simulink model "microgrid_case5"  (R2026a)
settings: Solver=ode14x  FixedStep=50e-6
libraries: ee_lib x65, nesl_utility x33, fl_lib x29, simulink x2
(part 1 of 2)
settings Model: Creator=HAKAN SARI  LastModifiedBy=HAKAN SARI

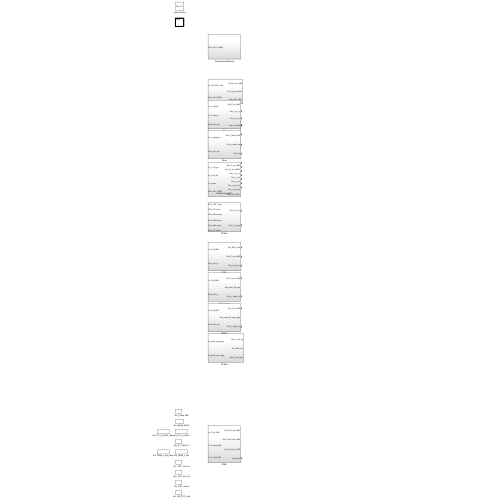
[thumbnail: Simulink's stored preview of the top-level diagram]
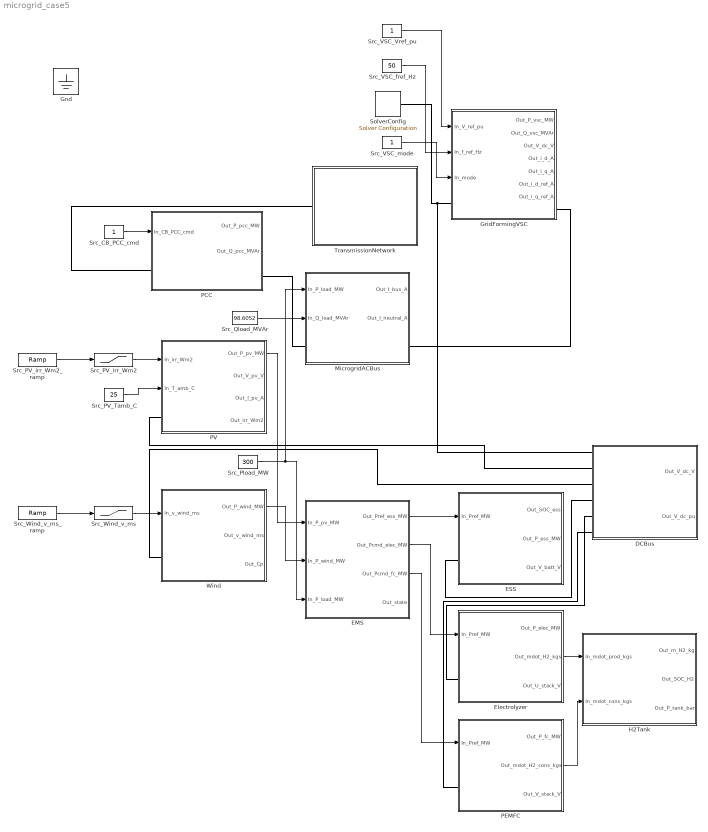
== system microgrid_case5 ==
  DCBus : Subsystem
  EMS : Subsystem
  ESS : Subsystem
  Electrolyzer : Subsystem
  Gnd : fl_lib/Electrical/Electrical Elements/Electrical Reference
  GridFormingVSC : Subsystem
  H2Tank : Subsystem
  MicrogridACBus : Subsystem
  PCC : Subsystem
  PEMFC : Subsystem
  PV : Subsystem
  SolverConfig : nesl_utility/Solver Configuration  PhysicalDomain=network_engine_domain  SubClassName=solver  LeftPortType=input  RightPortType=generic  Tones=[]  Harmonics=[]  SimulateNoise=off  Profile=off  UseLocalSampling=off  EnableSwitchedLinearOptims=on  FrequencyDomain=off  UseCCode=off  RelTol=0.001  AbsTol=0.001  MinStep=1e-09  ToWorkspace=off  RevertToSquareIcSolve=off  NumHomotopyIterations=100  PhasorMode=off  PhasorModeNumHarmonics=1  ConsistencySolver=NEWTON_XTOL_AFTER_FTOL  CanonicalOrdering=CANONICAL  OptimizeIntermediates=OPTIMIZED  IndexReductionMethod=DerivativeReplacement  DoDC=off  ResidualTolerance=1e-09  ConsistencyTolSource=GLOBAL  ConsistencyAbsTol=0.001  ConsistencyRelTol=0.001  ConsistencyTolFactor=0.001  UseLocalSolver=off  LocalSolverChoice=NE_BACKWARD_EULER_ADVANCER  ResolveIndetEquations=on  FunctionEvalNumThread=1  LocalSolverSampleTime=0.001  DoFixedCost=off  MaxNonlinIter=3  MaxModeIter=2  ComputeImpulses=off  ImpulseIterations=2  LinearAlgebra=auto  LinearAlgebraNumThread=0  EquationFormulation=NE_TIME_EF  DelaysMemoryBudget=1024  AutomaticFiltering=on  FilteringTimeConstant=0.001  PartitionStorageMethod=AS_NEEDED  PartitionMemoryBudget=1024  PartitionMethod=ROBUST  MultibodyUseLocalSolver=off  MultibodyLocalSolverChoice=ODE1  MultibodyLocalSolverSampleTime=0.001
  Src_CB_PCC_cmd : Constant
  Src_PV_Tamb_C : Constant  Value=25
  Src_PV_irr_Wm2 : Saturate  UpperLimit=800  LowerLimit=0
  Src_PV_irr_Wm2_ramp : simulink/Sources/Ramp  slope=800  start=0  InitialOutput=0
  Src_Pload_MW : Constant  Value=300
  Src_Qload_MVAr : Constant  Value=98.6052
  Src_VSC_Vref_pu : Constant
  Src_VSC_fref_Hz : Constant  Value=50
  Src_VSC_mode : Constant
  Src_Wind_v_ms : Saturate  UpperLimit=9  LowerLimit=0
  Src_Wind_v_ms_ramp : simulink/Sources/Ramp  slope=9  start=0  InitialOutput=0
  TransmissionNetwork : Subsystem
  Wind : Subsystem
  wires:
  Src_Wind_v_ms/1 -> Wind/1(In_v_wind_ms)
  Src_PV_irr_Wm2_ramp/1 -> Src_PV_irr_Wm2/1
  Src_VSC_mode/1 -> GridFormingVSC/3(In_mode)
  Src_Wind_v_ms_ramp/1 -> Src_Wind_v_ms/1
  Src_CB_PCC_cmd/1 -> PCC/1(In_CB_PCC_cmd)
  Src_PV_irr_Wm2/1 -> PV/1(In_irr_Wm2)
  Src_PV_Tamb_C/1 -> PV/2(In_T_amb_C)
  EMS/3(Out_Pcmd_fc_MW) -> PEMFC/1(In_Pref_MW)
  Src_Qload_MVAr/1 -> MicrogridACBus/2(In_Q_load_MVAr)
  PV/1(Out_P_pv_MW) -> EMS/1(In_P_pv_MW)
  Src_Pload_MW/1 -> MicrogridACBus/1(In_P_load_MW), EMS/3(In_P_load_MW)
  Wind/1(Out_P_wind_MW) -> EMS/2(In_P_wind_MW)
  Src_VSC_Vref_pu/1 -> GridFormingVSC/1(In_V_ref_pu)
  Src_VSC_fref_Hz/1 -> GridFormingVSC/2(In_f_ref_Hz)
  EMS/1(Out_Pref_ess_MW) -> ESS/1(In_Pref_MW)
  EMS/2(Out_Pcmd_elec_MW) -> Electrolyzer/1(In_Pref_MW)
  Electrolyzer/2(Out_mdot_H2_kgs) -> H2Tank/1(In_mdot_prod_kgs)
  PEMFC/2(Out_mdot_H2_cons_kgs) -> H2Tank/2(In_mdot_cons_kgs)
  connections:
  PEMFC/LConn1 -- DCBus/LConn6
  PV/LConn1 -- DCBus/LConn2
  MicrogridACBus/RConn1 -- GridFormingVSC/RConn1
  Wind/LConn1 -- DCBus/LConn3
  PCC/RConn1 -- MicrogridACBus/LConn1
  TransmissionNetwork/LConn1 -- PCC/LConn1
  SolverConfig/RConn1 -- GridFormingVSC/LConn1 -- DCBus/LConn1
  ESS/LConn1 -- DCBus/LConn4
  Electrolyzer/LConn1 -- DCBus/LConn5

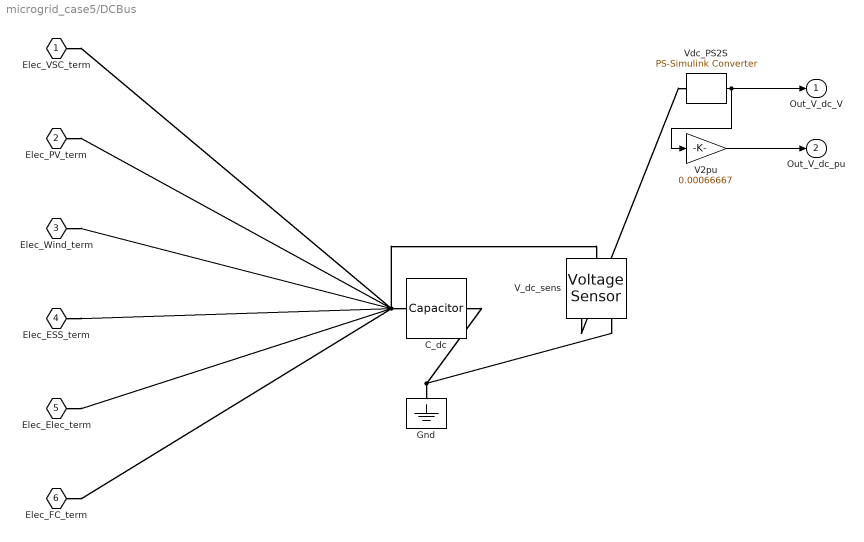
== system microgrid_case5/DCBus ==
  C_dc : ee_lib/Passive/Capacitor  cap_option=ee.enum.passive.capacitor.capOption.const  c=0.03 F  Cvec=[1e-05, 1e-06] F  Vvec=[0, 10] V  CV_table_symmetry=ee.enum.passive.capacitor.tableSymmetry.yes  f_vec=[1, 10] kHz  DFext_vec=[.8, 1.2]  enable_C_tol=ee.enum.toleranceApplication.none  averaging_period=0 s  C_tol=5  tol_distribution=ee.enum.toleranceDistribution.uniform  nSigma=4  r=0.001 Ohm  g=0 1/Ohm  enable_operating_limits=ee.enum.enable.no  operating_limit_action=ee.enum.passive.reportOpLim.warn  max_working_voltage_range=[-25, 25] V  power_rating=1 W  maxTemperature=85 degC  thermalEnable=false  thermalMass=1 J/K  i_specify=off  i_priority=None  i=0 A  i_nominal_specify=off  i_nominal_value=1  i_nominal_unit=A  v_specify=off  v_priority=None  v=0 V  v_nominal_specify=off  v_nominal_value=1  v_nominal_unit=V  vc_specify=on  vc_priority=High  vc=1500 V  vc_nominal_specify=off  vc_nominal_value=1  vc_nominal_unit=V  T_specify=off  T_priority=None  T=298.15 K  T_nominal_specify=off  T_nominal_value=1  T_nominal_unit=K
  Gnd : fl_lib/Electrical/Electrical Elements/Electrical Reference
  V2pu : Gain  Gain=0.00066667
  V_dc_sens : fl_lib/Electrical/Electrical Sensors/Voltage Sensor
  Vdc_PS2S : nesl_utility/PS-Simulink Converter  PhysicalDomain=network_engine_domain  SubClassName=ps_output  LeftPortType=input  RightPortType=output  PseudoPeriodic=off  Frequencies=[]  VectorFormat=inherit  Unit=V  AffineConversion=off
  Elec_VSC_term : PMIOPort  Side=Left
  Elec_PV_term : PMIOPort  Port=2  Side=Left
  Elec_Wind_term : PMIOPort  Port=3  Side=Left
  Elec_ESS_term : PMIOPort  Port=4  Side=Left
  Elec_Elec_term : PMIOPort  Port=5  Side=Left
  Elec_FC_term : PMIOPort  Port=6  Side=Left
  Out_V_dc_V : Outport
  Out_V_dc_pu : Outport  Port=2
  wires:
  Vdc_PS2S/1 -> Out_V_dc_V/1, V2pu/1
  V2pu/1 -> Out_V_dc_pu/1
  connections:
  Gnd/LConn1 -- C_dc/RConn1 -- V_dc_sens/RConn2
  Elec_VSC_term/RConn1 -- Elec_PV_term/RConn1 -- Elec_Wind_term/RConn1 -- Elec_ESS_term/RConn1 -- Elec_Elec_term/RConn1 -- Elec_FC_term/RConn1 -- C_dc/LConn1 -- V_dc_sens/LConn1
  V_dc_sens/RConn1 -- Vdc_PS2S/LConn1

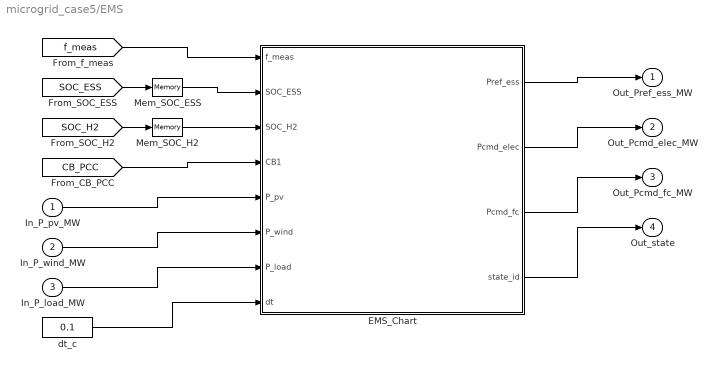
== system microgrid_case5/EMS ==
  In_P_pv_MW : Inport
  In_P_wind_MW : Inport  Port=2
  In_P_load_MW : Inport  Port=3
  EMS_Chart : Stateflow chart  TreatAsAtomicUnit=on
  Mem_SOC_ESS : Memory  InitialCondition=0.6
  Mem_SOC_H2 : Memory  InitialCondition=0.5
  dt_c : Constant  Value=0.1
  Out_Pref_ess_MW : Outport
  Out_Pcmd_elec_MW : Outport  Port=2
  Out_Pcmd_fc_MW : Outport  Port=3
  Out_state : Outport  Port=4
  wires:
  [f_meas] -> EMS_Chart/1(f_meas)
  [SOC_ESS] -> Mem_SOC_ESS/1
  Mem_SOC_ESS/1 -> EMS_Chart/2(SOC_ESS)
  [SOC_H2] -> Mem_SOC_H2/1
  Mem_SOC_H2/1 -> EMS_Chart/3(SOC_H2)
  [CB_PCC] -> EMS_Chart/4(CB1)
  In_P_pv_MW/1 -> EMS_Chart/5(P_pv)
  In_P_wind_MW/1 -> EMS_Chart/6(P_wind)
  In_P_load_MW/1 -> EMS_Chart/7(P_load)
  dt_c/1 -> EMS_Chart/8(dt)
  EMS_Chart/1(Pref_ess) -> Out_Pref_ess_MW/1
  EMS_Chart/2(Pcmd_elec) -> Out_Pcmd_elec_MW/1
  EMS_Chart/3(Pcmd_fc) -> Out_Pcmd_fc_MW/1
  EMS_Chart/4(state_id) -> Out_state/1

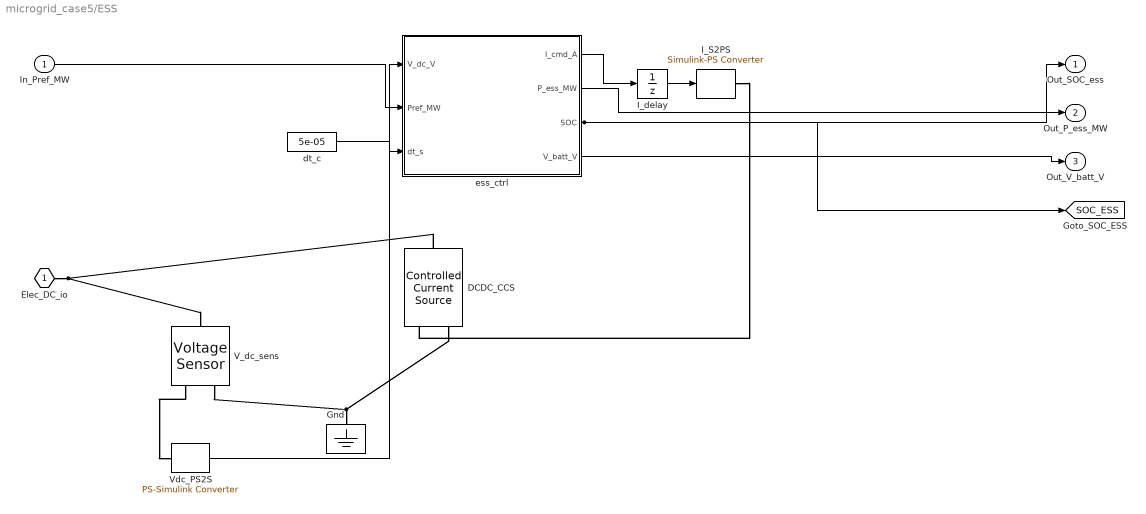
== system microgrid_case5/ESS ==
  In_Pref_MW : Inport
  DCDC_CCS : fl_lib/Electrical/Electrical Sources/Controlled Current Source
  Gnd : fl_lib/Electrical/Electrical Elements/Electrical Reference
  I_S2PS : nesl_utility/Simulink-PS Converter  PhysicalDomain=network_engine_domain  SubClassName=ps_input  LeftPortType=input  RightPortType=output  PseudoPeriodic=off  Frequencies=[]  NoiseDistribution=none  NoiseParameters=[]  Unit=A  AffineConversion=off  FilteringAndDerivatives=filter  SimscapeFilterOrder=1  InputFilterTimeConstant=1e-4  UdotUserProvided=0
  I_delay : UnitDelay  SampleTime=5e-05
  V_dc_sens : fl_lib/Electrical/Electrical Sensors/Voltage Sensor
  Vdc_PS2S : nesl_utility/PS-Simulink Converter  PhysicalDomain=network_engine_domain  SubClassName=ps_output  LeftPortType=input  RightPortType=output  PseudoPeriodic=off  Frequencies=[]  VectorFormat=inherit  Unit=V  AffineConversion=off
  dt_c : Constant  Value=5e-05
  ess_ctrl : MATLAB Function  TreatAsAtomicUnit=on
  Elec_DC_io : PMIOPort  Side=Left
  Out_SOC_ess : Outport
  Out_P_ess_MW : Outport  Port=2
  Out_V_batt_V : Outport  Port=3
  tag scope: SOC_ESS=global
  wires:
  Vdc_PS2S/1 -> ess_ctrl/1(V_dc_V)
  In_Pref_MW/1 -> ess_ctrl/2(Pref_MW)
  dt_c/1 -> ess_ctrl/3(dt_s)
  ess_ctrl/1(I_cmd_A) -> I_delay/1
  I_delay/1 -> I_S2PS/1
  ess_ctrl/2(P_ess_MW) -> Out_P_ess_MW/1
  ess_ctrl/3(SOC) -> Out_SOC_ess/1, [SOC_ESS]
  ess_ctrl/4(V_batt_V) -> Out_V_batt_V/1
  connections:
  V_dc_sens/LConn1 -- Elec_DC_io/RConn1 -- DCDC_CCS/LConn1
  Gnd/LConn1 -- V_dc_sens/RConn2 -- DCDC_CCS/RConn2
  V_dc_sens/RConn1 -- Vdc_PS2S/LConn1
  I_S2PS/RConn1 -- DCDC_CCS/RConn1

== system microgrid_case5/Electrolyzer ==
  In_Pref_MW : Inport
  EL_CCS : fl_lib/Electrical/Electrical Sources/Controlled Current Source
  Gnd : fl_lib/Electrical/Electrical Elements/Electrical Reference
  I_S2PS : nesl_utility/Simulink-PS Converter  PhysicalDomain=network_engine_domain  SubClassName=ps_input  LeftPortType=input  RightPortType=output  PseudoPeriodic=off  Frequencies=[]  NoiseDistribution=none  NoiseParameters=[]  Unit=A  AffineConversion=off  FilteringAndDerivatives=filter  SimscapeFilterOrder=1  InputFilterTimeConstant=1e-4  UdotUserProvided=0
  I_delay : UnitDelay  SampleTime=5e-05
  V_dc_sens : fl_lib/Electrical/Electrical Sensors/Voltage Sensor
  Vdc_PS2S : nesl_utility/PS-Simulink Converter  PhysicalDomain=network_engine_domain  SubClassName=ps_output  LeftPortType=input  RightPortType=output  PseudoPeriodic=off  Frequencies=[]  VectorFormat=inherit  Unit=V  AffineConversion=off
  dt_c : Constant  Value=5e-05
  el_ctrl : MATLAB Function  TreatAsAtomicUnit=on
  Elec_DC_in : PMIOPort  Side=Left
  Out_P_elec_MW : Outport
  Out_mdot_H2_kgs : Outport  Port=2
  Out_U_stack_V : Outport  Port=3
  wires:
  In_Pref_MW/1 -> el_ctrl/1(Pref_MW)
  Vdc_PS2S/1 -> el_ctrl/2(V_dc_V)
  dt_c/1 -> el_ctrl/3(dt_s)
  el_ctrl/2(P_elec_MW) -> Out_P_elec_MW/1
  el_ctrl/3(mdot_H2_kgs) -> Out_mdot_H2_kgs/1
  el_ctrl/4(U_stack_V) -> Out_U_stack_V/1
  el_ctrl/1(I_cmd_A) -> I_delay/1
  I_delay/1 -> I_S2PS/1
  connections:
  V_dc_sens/LConn1 -- Elec_DC_in/RConn1 -- EL_CCS/LConn1
  Gnd/LConn1 -- V_dc_sens/RConn2 -- EL_CCS/RConn2
  V_dc_sens/RConn1 -- Vdc_PS2S/LConn1
  I_S2PS/RConn1 -- EL_CCS/RConn1

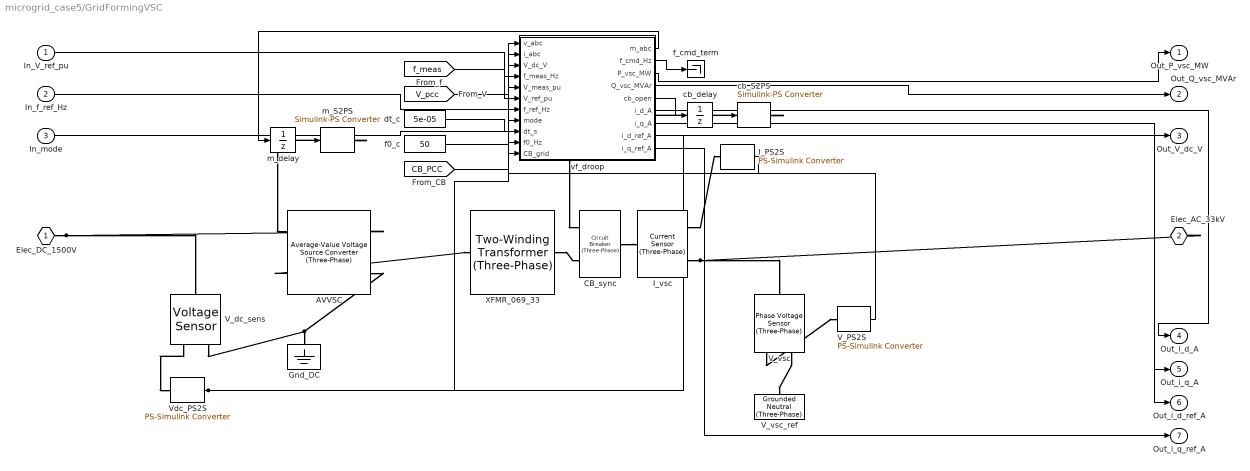
== system microgrid_case5/GridFormingVSC ==
  In_V_ref_pu : Inport
  In_f_ref_Hz : Inport  Port=2
  In_mode : Inport  Port=3
  AVVSC : ee_lib/Semiconductors & Converters/Converters/Average-Value Voltage Source Converter (Three-Phase)  port_option=ee.enum.threePhasePort.composite  enable_block_pulses_input=false  krec=0.01 Ohm  frequency_option=ee.enum.converters.frequency.variable  input_option=ee.enum.converters.inputOption.ModWave  FRated=50 Hz  losses_parameterization=ee.enum.converters.losses.fixed  Pfixed=1 W  ks=0.01  kc1=1.7 V  kc2=0.01 Ohm  Ploss_vect=[100, 800, 1870, 3250, 4900] W  Irms_vect=[10, 100, 200, 300, 400] A  Vdc_nom=1500 V  thermal_mass=30000 J/K  temperature_specify=off  temperature_priority=High  temperature=298.15 K  temperature_nominal_specify=off  temperature_nominal_value=1  temperature_nominal_unit=K
  CB_sync : ee_lib/Switches & Breakers/Circuit Breaker (Three-Phase)  port_option=ee.enum.threePhasePort.composite  control_port_option=ee.enum.controlport.ps  R_closed=1e-3 Ohm  G_open=1e-6 1/Ohm  threshold=0.5 V  breaker_behavior=ee.enum.switches.breakerBehavior.zeroCrossingEnable  i_th=1e-8 A
  Gnd_DC : fl_lib/Electrical/Electrical Elements/Electrical Reference
  I_PS2S : nesl_utility/PS-Simulink Converter  PhysicalDomain=network_engine_domain  SubClassName=ps_output  LeftPortType=input  RightPortType=output  PseudoPeriodic=off  Frequencies=[]  VectorFormat=inherit  Unit=inherit  AffineConversion=off
  I_vsc : ee_lib/Sensors & Transducers/Current Sensor (Three-Phase)  port_option=ee.enum.threePhasePort.composite
  V_PS2S : nesl_utility/PS-Simulink Converter  PhysicalDomain=network_engine_domain  SubClassName=ps_output  LeftPortType=input  RightPortType=output  PseudoPeriodic=off  Frequencies=[]  VectorFormat=inherit  Unit=inherit  AffineConversion=off
  V_dc_sens : fl_lib/Electrical/Electrical Sensors/Voltage Sensor
  V_vsc : ee_lib/Sensors & Transducers/Phase Voltage Sensor (Three-Phase)  port_option=ee.enum.threePhasePort.composite
  V_vsc_ref : ee_lib/Connectors & References/Grounded Neutral (Three-Phase)  port_option=ee.enum.threePhasePort.composite
  Vdc_PS2S : nesl_utility/PS-Simulink Converter  PhysicalDomain=network_engine_domain  SubClassName=ps_output  LeftPortType=input  RightPortType=output  PseudoPeriodic=off  Frequencies=[]  VectorFormat=inherit  Unit=V  AffineConversion=off
  XFMR_069_33 : ee_lib/Passive/Transformers/Two-Winding Transformer (Three-Phase)  SRated=350000000 A*V  FRated=50 Hz  Winding1Connection=ee.enum.windingconnection.Yg  VRated1=690 V  Winding2Connection=ee.enum.windingconnection.delta11  VRated2=33000 V  CoreType=ee.enum.coretype.threelimb  pu_Rw1=0.002  pu_Rw2=0.002  leakage_reactance_option=ee.enum.transformer_leakage.include  pu_Xl1=0.05  pu_Xl2=0.05  magnetizing_resistance_option=ee.enum.transformer_magnetizingResistance.exclude  pu_Rm=500  magnetizing_reactance_option=ee.enum.transformer_magnetizingReactance.exclude  saturation_option=ee.enum.transformer_saturation.exclude  pu_Xm=500  current_data=[0, .002, 1, 2]  magnetic_flux_data=[0, 1.2, 1.5, 1.51]  pu_X0=0.5  i1_specify=off  i1_priority=None  i1=[0, 0, 0] A  i1_nominal_specify=off  i1_nominal_value=1  i1_nominal_unit=A  i2_specify=off  i2_priority=None  i2=[0, 0, 0] A  i2_nominal_specify=off  i2_nominal_value=1  i2_nominal_unit=A  phi_specify=off  phi_priority=None  phi=[0, 0, 0]  phi_nominal_specify=off  phi_nominal_value=1  phi_nominal_unit=1
  cb_S2PS : nesl_utility/Simulink-PS Converter  PhysicalDomain=network_engine_domain  SubClassName=ps_input  LeftPortType=input  RightPortType=output  PseudoPeriodic=off  Frequencies=[]  NoiseDistribution=none  NoiseParameters=[]  Unit=1  AffineConversion=off  FilteringAndDerivatives=provide  SimscapeFilterOrder=1  InputFilterTimeConstant=0.001  UdotUserProvided=0
  cb_delay : UnitDelay  InitialCondition=1  SampleTime=5e-05
  dt_c : Constant  Value=5e-05
  f0_c : Constant  Value=50
  f_cmd_term : Terminator
  m_S2PS : nesl_utility/Simulink-PS Converter  PhysicalDomain=network_engine_domain  SubClassName=ps_input  LeftPortType=input  RightPortType=output  PseudoPeriodic=off  Frequencies=[]  NoiseDistribution=none  NoiseParameters=[]  Unit=1  AffineConversion=off  FilteringAndDerivatives=filter  SimscapeFilterOrder=1  InputFilterTimeConstant=1e-4  UdotUserProvided=0
  m_delay : UnitDelay  SampleTime=5e-05
  vf_droop : MATLAB Function  TreatAsAtomicUnit=on
  Elec_DC_1500V : PMIOPort  Side=Left
  Elec_AC_33kV : PMIOPort  Port=2  Side=Right
  Out_P_vsc_MW : Outport
  Out_Q_vsc_MVAr : Outport  Port=2
  Out_V_dc_V : Outport  Port=3
  Out_i_d_A : Outport  Port=4
  Out_i_q_A : Outport  Port=5
  Out_i_d_ref_A : Outport  Port=6
  Out_i_q_ref_A : Outport  Port=7
  wires:
  Vdc_PS2S/1 -> Out_V_dc_V/1, vf_droop/3(V_dc_V)
  V_PS2S/1 -> vf_droop/1(v_abc)
  I_PS2S/1 -> vf_droop/2(i_abc)
  [f_meas] -> vf_droop/4(f_meas_Hz)
  [V_pcc] -> vf_droop/5(V_meas_pu)
  In_V_ref_pu/1 -> vf_droop/6(V_ref_pu)
  In_f_ref_Hz/1 -> vf_droop/7(f_ref_Hz)
  In_mode/1 -> vf_droop/8(mode)
  dt_c/1 -> vf_droop/9(dt_s)
  f0_c/1 -> vf_droop/10(f0_Hz)
  [CB_PCC] -> vf_droop/11(CB_grid)
  vf_droop/1(m_abc) -> m_delay/1
  m_delay/1 -> m_S2PS/1
  vf_droop/2(f_cmd_Hz) -> f_cmd_term/1
  vf_droop/3(P_vsc_MW) -> Out_P_vsc_MW/1
  vf_droop/4(Q_vsc_MVAr) -> Out_Q_vsc_MVAr/1
  vf_droop/6(i_d_A) -> Out_i_d_A/1
  vf_droop/7(i_q_A) -> Out_i_q_A/1
  vf_droop/8(i_d_ref_A) -> Out_i_d_ref_A/1
  vf_droop/9(i_q_ref_A) -> Out_i_q_ref_A/1
  vf_droop/5(cb_open) -> cb_delay/1
  cb_delay/1 -> cb_S2PS/1
  connections:
  AVVSC/RConn1 -- Elec_DC_1500V/RConn1 -- V_dc_sens/LConn1
  Gnd_DC/LConn1 -- AVVSC/RConn2 -- V_dc_sens/RConn2
  V_dc_sens/RConn1 -- Vdc_PS2S/LConn1
  AVVSC/LConn2 -- XFMR_069_33/LConn1
  XFMR_069_33/RConn1 -- CB_sync/LConn2
  CB_sync/RConn1 -- I_vsc/LConn1
  Elec_AC_33kV/RConn1 -- I_vsc/RConn2 -- V_vsc/LConn1
  V_vsc/RConn2 -- V_vsc_ref/LConn1
  I_vsc/RConn1 -- I_PS2S/LConn1
  V_vsc/RConn1 -- V_PS2S/LConn1
  m_S2PS/RConn1 -- AVVSC/LConn1
  cb_S2PS/RConn1 -- CB_sync/LConn1

== system microgrid_case5/H2Tank ==
  In_mdot_prod_kgs : Inport
  In_mdot_cons_kgs : Inport  Port=2
  dt_c : Constant  Value=5e-05
  tank_dynamics : MATLAB Function  TreatAsAtomicUnit=on
  Out_m_H2_kg : Outport
  Out_SOC_H2 : Outport  Port=2
  Out_P_tank_bar : Outport  Port=3
  tag scope: SOC_H2=global
  wires:
  In_mdot_prod_kgs/1 -> tank_dynamics/1(mdot_prod_kgs)
  In_mdot_cons_kgs/1 -> tank_dynamics/2(mdot_cons_kgs)
  dt_c/1 -> tank_dynamics/3(dt_s)
  tank_dynamics/1(m_H2_kg) -> Out_m_H2_kg/1
  tank_dynamics/2(SOC_H2) -> Out_SOC_H2/1, [SOC_H2]
  tank_dynamics/3(P_tank_bar) -> Out_P_tank_bar/1

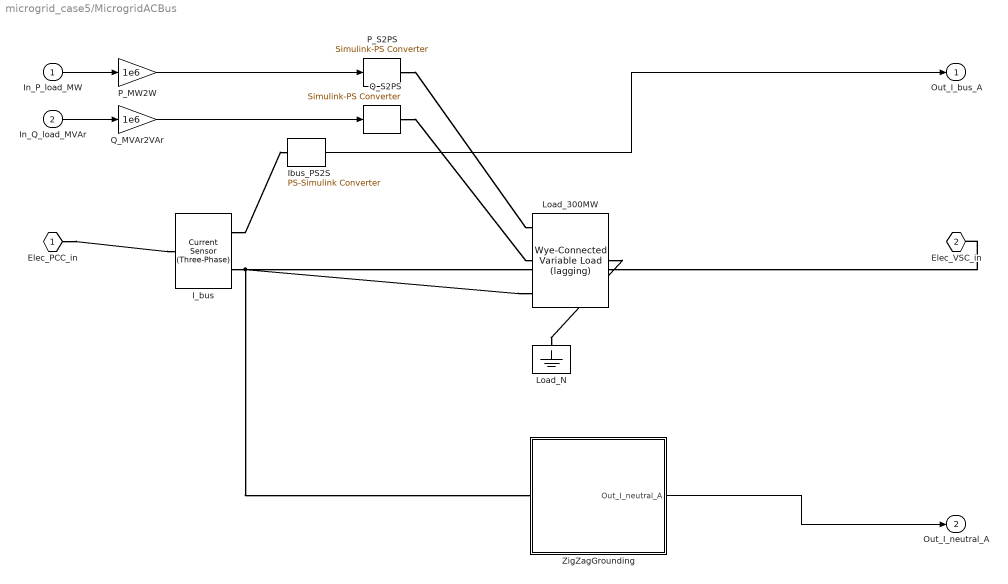
== system microgrid_case5/MicrogridACBus ==
  In_P_load_MW : Inport
  In_Q_load_MVAr : Inport  Port=2
  I_bus : ee_lib/Sensors & Transducers/Current Sensor (Three-Phase)  port_option=ee.enum.threePhasePort.composite
  Ibus_PS2S : nesl_utility/PS-Simulink Converter  PhysicalDomain=network_engine_domain  SubClassName=ps_output  LeftPortType=input  RightPortType=output  PseudoPeriodic=off  Frequencies=[]  VectorFormat=inherit  Unit=inherit  AffineConversion=off
  Load_300MW : ee_lib/Passive/RLC Assemblies/Wye-Connected Variable Load (lagging)  port_option=ee.enum.threePhasePort.composite  VRated=33000 V  FRated=50 Hz  Pmin=1e3 W  Qmin=1e3 A*V  G_parasitic=1e-6 1/Ohm  I_specify=off  I_priority=None  I=[0, 0, 0] A  I_nominal_specify=off  I_nominal_value=1  I_nominal_unit=A  Phi_specify=off  Phi_priority=None  Phi=[0, 0, 0] Wb  Phi_nominal_specify=off  Phi_nominal_value=1  Phi_nominal_unit=Wb
  Load_N : fl_lib/Electrical/Electrical Elements/Electrical Reference
  P_MW2W : Gain  Gain=1e6
  P_S2PS : nesl_utility/Simulink-PS Converter  PhysicalDomain=network_engine_domain  SubClassName=ps_input  LeftPortType=input  RightPortType=output  PseudoPeriodic=off  Frequencies=[]  NoiseDistribution=none  NoiseParameters=[]  Unit=W  AffineConversion=off  FilteringAndDerivatives=provide  SimscapeFilterOrder=1  InputFilterTimeConstant=0.001  UdotUserProvided=0
  Q_MVAr2VAr : Gain  Gain=1e6
  Q_S2PS : nesl_utility/Simulink-PS Converter  PhysicalDomain=network_engine_domain  SubClassName=ps_input  LeftPortType=input  RightPortType=output  PseudoPeriodic=off  Frequencies=[]  NoiseDistribution=none  NoiseParameters=[]  Unit=V*A  AffineConversion=off  FilteringAndDerivatives=provide  SimscapeFilterOrder=1  InputFilterTimeConstant=0.001  UdotUserProvided=0
  ZigZagGrounding : Subsystem
  Elec_PCC_in : PMIOPort  Side=Left
  Elec_VSC_in : PMIOPort  Port=2  Side=Right
  Out_I_bus_A : Outport
  Out_I_neutral_A : Outport  Port=2
  wires:
  Ibus_PS2S/1 -> Out_I_bus_A/1
  In_P_load_MW/1 -> P_MW2W/1
  P_MW2W/1 -> P_S2PS/1
  In_Q_load_MVAr/1 -> Q_MVAr2VAr/1
  Q_MVAr2VAr/1 -> Q_S2PS/1
  ZigZagGrounding/1(Out_I_neutral_A) -> Out_I_neutral_A/1
  connections:
  Elec_PCC_in/RConn1 -- I_bus/LConn1
  I_bus/RConn1 -- Ibus_PS2S/LConn1
  Load_300MW/LConn3 -- I_bus/RConn2 -- Elec_VSC_in/RConn1 -- ZigZagGrounding/LConn1
  Load_300MW/RConn1 -- Load_N/LConn1
  P_S2PS/RConn1 -- Load_300MW/LConn1
  Q_S2PS/RConn1 -- Load_300MW/LConn2

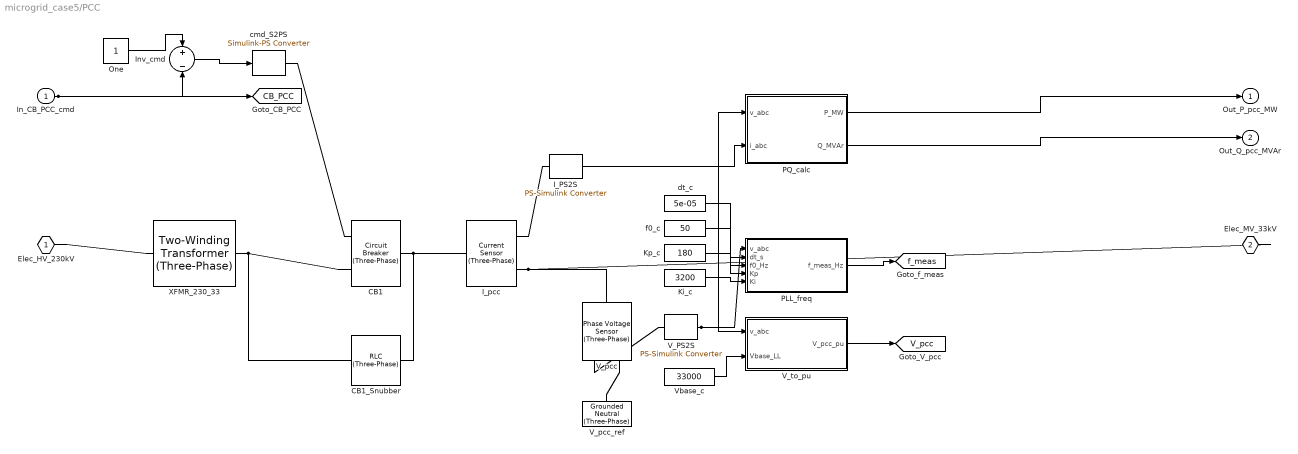
== system microgrid_case5/PCC ==
  In_CB_PCC_cmd : Inport
  CB1 : ee_lib/Switches & Breakers/Circuit Breaker (Three-Phase)  port_option=ee.enum.threePhasePort.composite  control_port_option=ee.enum.controlport.ps  R_closed=1e-3 Ohm  G_open=1e-6 1/Ohm  threshold=0.5 V  breaker_behavior=ee.enum.switches.breakerBehavior.zeroCrossingEnable  i_th=1e-8 A
  CB1_Snubber : ee_lib/Passive/RLC Assemblies/RLC (Three-Phase)  port_option=ee.enum.threePhasePort.composite  component_structure=ee.enum.rlc.structure.SeriesRC  R=200 Ohm  L=1e-3 H  C=1e-06 F  R_parasitic=0 Ohm  G_parasitic=0 1/Ohm  IL_specify=off  IL_priority=High  IL=[0, 0, 0] A  IL_nominal_specify=off  IL_nominal_value=1  IL_nominal_unit=A  VC_specify=off  VC_priority=High  VC=[0, 0, 0] V  VC_nominal_specify=off  VC_nominal_value=1  VC_nominal_unit=V
  I_PS2S : nesl_utility/PS-Simulink Converter  PhysicalDomain=network_engine_domain  SubClassName=ps_output  LeftPortType=input  RightPortType=output  PseudoPeriodic=off  Frequencies=[]  VectorFormat=inherit  Unit=inherit  AffineConversion=off
  I_pcc : ee_lib/Sensors & Transducers/Current Sensor (Three-Phase)  port_option=ee.enum.threePhasePort.composite
  Inv_cmd : Sum  Inputs=+-
  Ki_c : Constant  Value=3200
  Kp_c : Constant  Value=180
  One : Constant
  PLL_freq : MATLAB Function  TreatAsAtomicUnit=on
  PQ_calc : MATLAB Function  TreatAsAtomicUnit=on
  V_PS2S : nesl_utility/PS-Simulink Converter  PhysicalDomain=network_engine_domain  SubClassName=ps_output  LeftPortType=input  RightPortType=output  PseudoPeriodic=off  Frequencies=[]  VectorFormat=inherit  Unit=inherit  AffineConversion=off
  V_pcc : ee_lib/Sensors & Transducers/Phase Voltage Sensor (Three-Phase)  port_option=ee.enum.threePhasePort.composite
  V_pcc_ref : ee_lib/Connectors & References/Grounded Neutral (Three-Phase)  port_option=ee.enum.threePhasePort.composite
  V_to_pu : MATLAB Function  TreatAsAtomicUnit=on
  Vbase_c : Constant  Value=33000
  XFMR_230_33 : ee_lib/Passive/Transformers/Two-Winding Transformer (Three-Phase)  SRated=300000000 A*V  FRated=50 Hz  Winding1Connection=ee.enum.windingconnection.delta11  VRated1=230000 V  Winding2Connection=ee.enum.windingconnection.Yg  VRated2=33000 V  CoreType=ee.enum.coretype.threelimb  pu_Rw1=0.002  pu_Rw2=0.002  leakage_reactance_option=ee.enum.transformer_leakage.include  pu_Xl1=0.05  pu_Xl2=0.05  magnetizing_resistance_option=ee.enum.transformer_magnetizingResistance.exclude  pu_Rm=500  magnetizing_reactance_option=ee.enum.transformer_magnetizingReactance.exclude  saturation_option=ee.enum.transformer_saturation.exclude  pu_Xm=500  current_data=[0, .002, 1, 2]  magnetic_flux_data=[0, 1.2, 1.5, 1.51]  pu_X0=0.5  i1_specify=off  i1_priority=None  i1=[0, 0, 0] A  i1_nominal_specify=off  i1_nominal_value=1  i1_nominal_unit=A  i2_specify=off  i2_priority=None  i2=[0, 0, 0] A  i2_nominal_specify=off  i2_nominal_value=1  i2_nominal_unit=A  phi_specify=off  phi_priority=None  phi=[0, 0, 0]  phi_nominal_specify=off  phi_nominal_value=1  phi_nominal_unit=1
  cmd_S2PS : nesl_utility/Simulink-PS Converter  PhysicalDomain=network_engine_domain  SubClassName=ps_input  LeftPortType=input  RightPortType=output  PseudoPeriodic=off  Frequencies=[]  NoiseDistribution=none  NoiseParameters=[]  Unit=1  AffineConversion=off  FilteringAndDerivatives=filter  SimscapeFilterOrder=1  InputFilterTimeConstant=1e-4  UdotUserProvided=0
  dt_c : Constant  Value=5e-05
  f0_c : Constant  Value=50
  Elec_HV_230kV : PMIOPort  Side=Left
  Elec_MV_33kV : PMIOPort  Port=2  Side=Right
  Out_P_pcc_MW : Outport
  Out_Q_pcc_MVAr : Outport  Port=2
  tag scope: CB_PCC=global, V_pcc=global, f_meas=global
  wires:
  One/1 -> Inv_cmd/1
  In_CB_PCC_cmd/1 -> Inv_cmd/2, [CB_PCC]
  Inv_cmd/1 -> cmd_S2PS/1
  V_PS2S/1 -> PLL_freq/1(v_abc), V_to_pu/1(v_abc), PQ_calc/1(v_abc)
  dt_c/1 -> PLL_freq/2(dt_s)
  f0_c/1 -> PLL_freq/3(f0_Hz)
  Kp_c/1 -> PLL_freq/4(Kp)
  Ki_c/1 -> PLL_freq/5(Ki)
  PLL_freq/1(f_meas_Hz) -> [f_meas]
  Vbase_c/1 -> V_to_pu/2(Vbase_LL)
  V_to_pu/1(V_pcc_pu) -> [V_pcc]
  I_PS2S/1 -> PQ_calc/2(i_abc)
  PQ_calc/1(P_MW) -> Out_P_pcc_MW/1
  PQ_calc/2(Q_MVAr) -> Out_Q_pcc_MVAr/1
  connections:
  Elec_HV_230kV/RConn1 -- XFMR_230_33/LConn1
  CB1/LConn2 -- XFMR_230_33/RConn1 -- CB1_Snubber/LConn1
  cmd_S2PS/RConn1 -- CB1/LConn1
  CB1_Snubber/RConn1 -- CB1/RConn1 -- I_pcc/LConn1
  Elec_MV_33kV/RConn1 -- I_pcc/RConn2 -- V_pcc/LConn1
  V_pcc/RConn2 -- V_pcc_ref/LConn1
  I_pcc/RConn1 -- I_PS2S/LConn1
  V_pcc/RConn1 -- V_PS2S/LConn1

== system microgrid_case5/PEMFC ==
  In_Pref_MW : Inport
  FC_CCS : fl_lib/Electrical/Electrical Sources/Controlled Current Source
  Gnd : fl_lib/Electrical/Electrical Elements/Electrical Reference
  I_S2PS : nesl_utility/Simulink-PS Converter  PhysicalDomain=network_engine_domain  SubClassName=ps_input  LeftPortType=input  RightPortType=output  PseudoPeriodic=off  Frequencies=[]  NoiseDistribution=none  NoiseParameters=[]  Unit=A  AffineConversion=off  FilteringAndDerivatives=filter  SimscapeFilterOrder=1  InputFilterTimeConstant=1e-4  UdotUserProvided=0
  I_delay : UnitDelay  SampleTime=5e-05
  V_dc_sens : fl_lib/Electrical/Electrical Sensors/Voltage Sensor
  Vdc_PS2S : nesl_utility/PS-Simulink Converter  PhysicalDomain=network_engine_domain  SubClassName=ps_output  LeftPortType=input  RightPortType=output  PseudoPeriodic=off  Frequencies=[]  VectorFormat=inherit  Unit=V  AffineConversion=off
  dt_c : Constant  Value=5e-05
  fc_ctrl : MATLAB Function  TreatAsAtomicUnit=on
  Elec_DC_out : PMIOPort  Side=Left
  Out_P_fc_MW : Outport
  Out_mdot_H2_cons_kgs : Outport  Port=2
  Out_V_stack_V : Outport  Port=3
  wires:
  In_Pref_MW/1 -> fc_ctrl/1(Pref_MW)
  Vdc_PS2S/1 -> fc_ctrl/2(V_dc_V)
  dt_c/1 -> fc_ctrl/3(dt_s)
  fc_ctrl/2(P_fc_MW) -> Out_P_fc_MW/1
  fc_ctrl/3(mdot_cons_kgs) -> Out_mdot_H2_cons_kgs/1
  fc_ctrl/4(V_stack_V) -> Out_V_stack_V/1
  fc_ctrl/1(I_cmd_A) -> I_delay/1
  I_delay/1 -> I_S2PS/1
  connections:
  V_dc_sens/LConn1 -- Elec_DC_out/RConn1 -- FC_CCS/LConn1
  Gnd/LConn1 -- V_dc_sens/RConn2 -- FC_CCS/RConn2
  V_dc_sens/RConn1 -- Vdc_PS2S/LConn1
  I_S2PS/RConn1 -- FC_CCS/RConn1

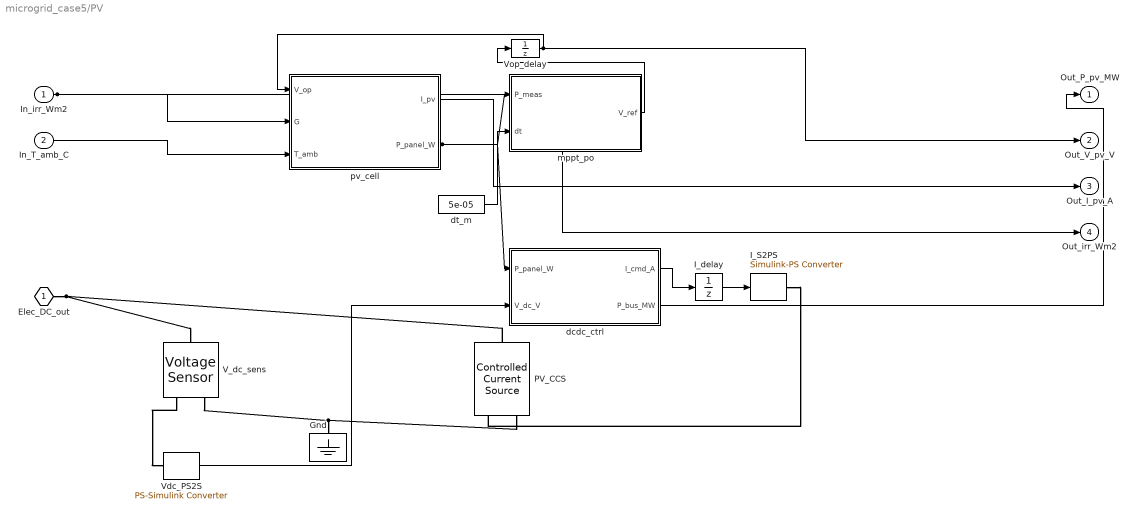
== system microgrid_case5/PV ==
  In_irr_Wm2 : Inport
  In_T_amb_C : Inport  Port=2
  Gnd : fl_lib/Electrical/Electrical Elements/Electrical Reference
  I_S2PS : nesl_utility/Simulink-PS Converter  PhysicalDomain=network_engine_domain  SubClassName=ps_input  LeftPortType=input  RightPortType=output  PseudoPeriodic=off  Frequencies=[]  NoiseDistribution=none  NoiseParameters=[]  Unit=A  AffineConversion=off  FilteringAndDerivatives=filter  SimscapeFilterOrder=1  InputFilterTimeConstant=1e-4  UdotUserProvided=0
  I_delay : UnitDelay  SampleTime=5e-05
  PV_CCS : fl_lib/Electrical/Electrical Sources/Controlled Current Source
  V_dc_sens : fl_lib/Electrical/Electrical Sensors/Voltage Sensor
  Vdc_PS2S : nesl_utility/PS-Simulink Converter  PhysicalDomain=network_engine_domain  SubClassName=ps_output  LeftPortType=input  RightPortType=output  PseudoPeriodic=off  Frequencies=[]  VectorFormat=inherit  Unit=V  AffineConversion=off
  Vop_delay : UnitDelay  InitialCondition=702  SampleTime=5e-05
  dcdc_ctrl : MATLAB Function  TreatAsAtomicUnit=on
  dt_m : Constant  Value=5e-05
  mppt_po : MATLAB Function  TreatAsAtomicUnit=on
  pv_cell : MATLAB Function  TreatAsAtomicUnit=on
  Elec_DC_out : PMIOPort  Side=Left
  Out_P_pv_MW : Outport
  Out_V_pv_V : Outport  Port=2
  Out_I_pv_A : Outport  Port=3
  Out_irr_Wm2 : Outport  Port=4
  wires:
  In_irr_Wm2/1 -> Out_irr_Wm2/1, pv_cell/2(G)
  In_T_amb_C/1 -> pv_cell/3(T_amb)
  pv_cell/2(P_panel_W) -> mppt_po/1(P_meas), dcdc_ctrl/1(P_panel_W)
  dt_m/1 -> mppt_po/2(dt)
  mppt_po/1(V_ref) -> Vop_delay/1
  Vop_delay/1 -> pv_cell/1(V_op), Out_V_pv_V/1
  pv_cell/1(I_pv) -> Out_I_pv_A/1
  Vdc_PS2S/1 -> dcdc_ctrl/2(V_dc_V)
  dcdc_ctrl/2(P_bus_MW) -> Out_P_pv_MW/1
  dcdc_ctrl/1(I_cmd_A) -> I_delay/1
  I_delay/1 -> I_S2PS/1
  connections:
  V_dc_sens/LConn1 -- Elec_DC_out/RConn1 -- PV_CCS/LConn1
  Gnd/LConn1 -- V_dc_sens/RConn2 -- PV_CCS/RConn2
  V_dc_sens/RConn1 -- Vdc_PS2S/LConn1
  I_S2PS/RConn1 -- PV_CCS/RConn1

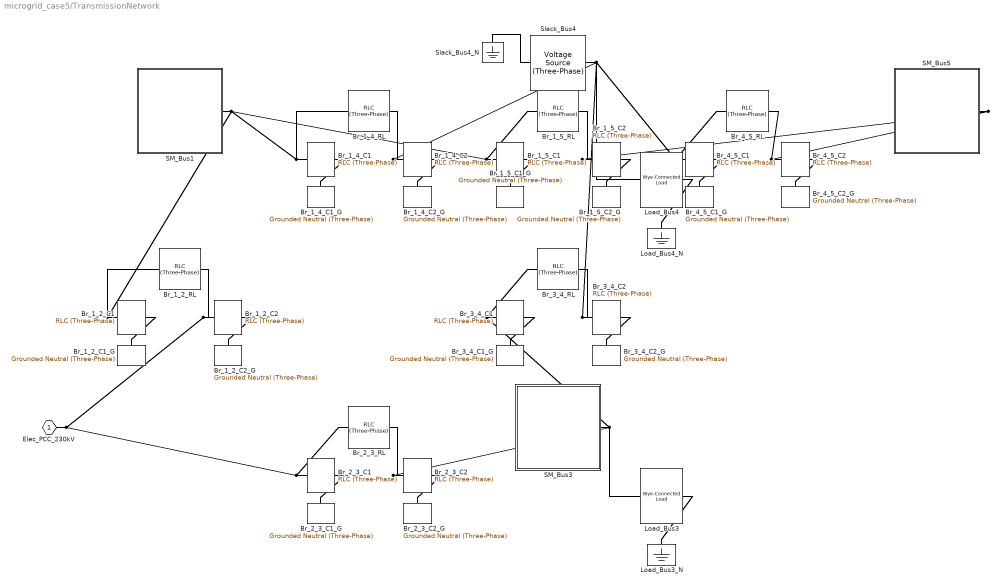
== system microgrid_case5/TransmissionNetwork ==
  Br_1_2_C1 : ee_lib/Passive/RLC Assemblies/RLC (Three-Phase)  port_option=ee.enum.threePhasePort.composite  component_structure=ee.enum.rlc.structure.C  R=1 Ohm  L=1e-3 H  C=2.1421e-08 F  R_parasitic=1 Ohm  G_parasitic=0 1/Ohm  IL_specify=off  IL_priority=High  IL=[0, 0, 0] A  IL_nominal_specify=off  IL_nominal_value=1  IL_nominal_unit=A  VC_specify=off  VC_priority=High  VC=[0, 0, 0] V  VC_nominal_specify=off  VC_nominal_value=1  VC_nominal_unit=V
  Br_1_2_C1_G : ee_lib/Connectors & References/Grounded Neutral (Three-Phase)  port_option=ee.enum.threePhasePort.composite
  Br_1_2_C2 : ee_lib/Passive/RLC Assemblies/RLC (Three-Phase)  port_option=ee.enum.threePhasePort.composite  component_structure=ee.enum.rlc.structure.C  R=1 Ohm  L=1e-3 H  C=2.1421e-08 F  R_parasitic=1 Ohm  G_parasitic=0 1/Ohm  IL_specify=off  IL_priority=High  IL=[0, 0, 0] A  IL_nominal_specify=off  IL_nominal_value=1  IL_nominal_unit=A  VC_specify=off  VC_priority=High  VC=[0, 0, 0] V  VC_nominal_specify=off  VC_nominal_value=1  VC_nominal_unit=V
  Br_1_2_C2_G : ee_lib/Connectors & References/Grounded Neutral (Three-Phase)  port_option=ee.enum.threePhasePort.composite
  Br_1_2_RL : ee_lib/Passive/RLC Assemblies/RLC (Three-Phase)  port_option=ee.enum.threePhasePort.composite  component_structure=ee.enum.rlc.structure.SeriesRL  R=1.4865 Ohm  L=0.047316 H  C=1e-6 F  R_parasitic=0 Ohm  G_parasitic=0 1/Ohm  IL_specify=off  IL_priority=High  IL=[0, 0, 0] A  IL_nominal_specify=off  IL_nominal_value=1  IL_nominal_unit=A  VC_specify=off  VC_priority=High  VC=[0, 0, 0] V  VC_nominal_specify=off  VC_nominal_value=1  VC_nominal_unit=V
  Br_1_4_C1 : ee_lib/Passive/RLC Assemblies/RLC (Three-Phase)  port_option=ee.enum.threePhasePort.composite  component_structure=ee.enum.rlc.structure.C  R=1 Ohm  L=1e-3 H  C=1.9797e-08 F  R_parasitic=1 Ohm  G_parasitic=0 1/Ohm  IL_specify=off  IL_priority=High  IL=[0, 0, 0] A  IL_nominal_specify=off  IL_nominal_value=1  IL_nominal_unit=A  VC_specify=off  VC_priority=High  VC=[0, 0, 0] V  VC_nominal_specify=off  VC_nominal_value=1  VC_nominal_unit=V
  Br_1_4_C1_G : ee_lib/Connectors & References/Grounded Neutral (Three-Phase)  port_option=ee.enum.threePhasePort.composite
  Br_1_4_C2 : ee_lib/Passive/RLC Assemblies/RLC (Three-Phase)  port_option=ee.enum.threePhasePort.composite  component_structure=ee.enum.rlc.structure.C  R=1 Ohm  L=1e-3 H  C=1.9797e-08 F  R_parasitic=1 Ohm  G_parasitic=0 1/Ohm  IL_specify=off  IL_priority=High  IL=[0, 0, 0] A  IL_nominal_specify=off  IL_nominal_value=1  IL_nominal_unit=A  VC_specify=off  VC_priority=High  VC=[0, 0, 0] V  VC_nominal_specify=off  VC_nominal_value=1  VC_nominal_unit=V
  Br_1_4_C2_G : ee_lib/Connectors & References/Grounded Neutral (Three-Phase)  port_option=ee.enum.threePhasePort.composite
  Br_1_4_RL : ee_lib/Passive/RLC Assemblies/RLC (Three-Phase)  port_option=ee.enum.threePhasePort.composite  component_structure=ee.enum.rlc.structure.SeriesRL  R=1.6082 Ohm  L=0.051189 H  C=1e-6 F  R_parasitic=0 Ohm  G_parasitic=0 1/Ohm  IL_specify=off  IL_priority=High  IL=[0, 0, 0] A  IL_nominal_specify=off  IL_nominal_value=1  IL_nominal_unit=A  VC_specify=off  VC_priority=High  VC=[0, 0, 0] V  VC_nominal_specify=off  VC_nominal_value=1  VC_nominal_unit=V
  Br_1_5_C1 : ee_lib/Passive/RLC Assemblies/RLC (Three-Phase)  port_option=ee.enum.threePhasePort.composite  component_structure=ee.enum.rlc.structure.C  R=1 Ohm  L=1e-3 H  C=9.4049e-08 F  R_parasitic=1 Ohm  G_parasitic=0 1/Ohm  IL_specify=off  IL_priority=High  IL=[0, 0, 0] A  IL_nominal_specify=off  IL_nominal_value=1  IL_nominal_unit=A  VC_specify=off  VC_priority=High  VC=[0, 0, 0] V  VC_nominal_specify=off  VC_nominal_value=1  VC_nominal_unit=V
  Br_1_5_C1_G : ee_lib/Connectors & References/Grounded Neutral (Three-Phase)  port_option=ee.enum.threePhasePort.composite
  Br_1_5_C2 : ee_lib/Passive/RLC Assemblies/RLC (Three-Phase)  port_option=ee.enum.threePhasePort.composite  component_structure=ee.enum.rlc.structure.C  R=1 Ohm  L=1e-3 H  C=9.4049e-08 F  R_parasitic=1 Ohm  G_parasitic=0 1/Ohm  IL_specify=off  IL_priority=High  IL=[0, 0, 0] A  IL_nominal_specify=off  IL_nominal_value=1  IL_nominal_unit=A  VC_specify=off  VC_priority=High  VC=[0, 0, 0] V  VC_nominal_specify=off  VC_nominal_value=1  VC_nominal_unit=V
  Br_1_5_C2_G : ee_lib/Connectors & References/Grounded Neutral (Three-Phase)  port_option=ee.enum.threePhasePort.composite
  Br_1_5_RL : ee_lib/Passive/RLC Assemblies/RLC (Three-Phase)  port_option=ee.enum.threePhasePort.composite  component_structure=ee.enum.rlc.structure.SeriesRL  R=0.33856 Ohm  L=0.010777 H  C=1e-6 F  R_parasitic=0 Ohm  G_parasitic=0 1/Ohm  IL_specify=off  IL_priority=High  IL=[0, 0, 0] A  IL_nominal_specify=off  IL_nominal_value=1  IL_nominal_unit=A  VC_specify=off  VC_priority=High  VC=[0, 0, 0] V  VC_nominal_specify=off  VC_nominal_value=1  VC_nominal_unit=V
  Br_2_3_C1 : ee_lib/Passive/RLC Assemblies/RLC (Three-Phase)  port_option=ee.enum.threePhasePort.composite  component_structure=ee.enum.rlc.structure.C  R=1 Ohm  L=1e-3 H  C=5.5719e-08 F  R_parasitic=1 Ohm  G_parasitic=0 1/Ohm  IL_specify=off  IL_priority=High  IL=[0, 0, 0] A  IL_nominal_specify=off  IL_nominal_value=1  IL_nominal_unit=A  VC_specify=off  VC_priority=High  VC=[0, 0, 0] V  VC_nominal_specify=off  VC_nominal_value=1  VC_nominal_unit=V
  Br_2_3_C1_G : ee_lib/Connectors & References/Grounded Neutral (Three-Phase)  port_option=ee.enum.threePhasePort.composite
  Br_2_3_C2 : ee_lib/Passive/RLC Assemblies/RLC (Three-Phase)  port_option=ee.enum.threePhasePort.composite  component_structure=ee.enum.rlc.structure.C  R=1 Ohm  L=1e-3 H  C=5.5719e-08 F  R_parasitic=1 Ohm  G_parasitic=0 1/Ohm  IL_specify=off  IL_priority=High  IL=[0, 0, 0] A  IL_nominal_specify=off  IL_nominal_value=1  IL_nominal_unit=A  VC_specify=off  VC_priority=High  VC=[0, 0, 0] V  VC_nominal_specify=off  VC_nominal_value=1  VC_nominal_unit=V
  Br_2_3_C2_G : ee_lib/Connectors & References/Grounded Neutral (Three-Phase)  port_option=ee.enum.threePhasePort.composite
  Br_2_3_RL : ee_lib/Passive/RLC Assemblies/RLC (Three-Phase)  port_option=ee.enum.threePhasePort.composite  component_structure=ee.enum.rlc.structure.SeriesRL  R=0.57132 Ohm  L=0.018186 H  C=1e-6 F  R_parasitic=0 Ohm  G_parasitic=0 1/Ohm  IL_specify=off  IL_priority=High  IL=[0, 0, 0] A  IL_nominal_specify=off  IL_nominal_value=1  IL_nominal_unit=A  VC_specify=off  VC_priority=High  VC=[0, 0, 0] V  VC_nominal_specify=off  VC_nominal_value=1  VC_nominal_unit=V
  Br_3_4_C1 : ee_lib/Passive/RLC Assemblies/RLC (Three-Phase)  port_option=ee.enum.threePhasePort.composite  component_structure=ee.enum.rlc.structure.C  R=1 Ohm  L=1e-3 H  C=2.0278e-08 F  R_parasitic=1 Ohm  G_parasitic=0 1/Ohm  IL_specify=off  IL_priority=High  IL=[0, 0, 0] A  IL_nominal_specify=off  IL_nominal_value=1  IL_nominal_unit=A  VC_specify=off  VC_priority=High  VC=[0, 0, 0] V  VC_nominal_specify=off  VC_nominal_value=1  VC_nominal_unit=V
  Br_3_4_C1_G : ee_lib/Connectors & References/Grounded Neutral (Three-Phase)  port_option=ee.enum.threePhasePort.composite
  Br_3_4_C2 : ee_lib/Passive/RLC Assemblies/RLC (Three-Phase)  port_option=ee.enum.threePhasePort.composite  component_structure=ee.enum.rlc.structure.C  R=1 Ohm  L=1e-3 H  C=2.0278e-08 F  R_parasitic=1 Ohm  G_parasitic=0 1/Ohm  IL_specify=off  IL_priority=High  IL=[0, 0, 0] A  IL_nominal_specify=off  IL_nominal_value=1  IL_nominal_unit=A  VC_specify=off  VC_priority=High  VC=[0, 0, 0] V  VC_nominal_specify=off  VC_nominal_value=1  VC_nominal_unit=V
  Br_3_4_C2_G : ee_lib/Connectors & References/Grounded Neutral (Three-Phase)  port_option=ee.enum.threePhasePort.composite
  Br_3_4_RL : ee_lib/Passive/RLC Assemblies/RLC (Three-Phase)  port_option=ee.enum.threePhasePort.composite  component_structure=ee.enum.rlc.structure.SeriesRL  R=1.5711 Ohm  L=0.050011 H  C=1e-6 F  R_parasitic=0 Ohm  G_parasitic=0 1/Ohm  IL_specify=off  IL_priority=High  IL=[0, 0, 0] A  IL_nominal_specify=off  IL_nominal_value=1  IL_nominal_unit=A  VC_specify=off  VC_priority=High  VC=[0, 0, 0] V  VC_nominal_specify=off  VC_nominal_value=1  VC_nominal_unit=V
  Br_4_5_C1 : ee_lib/Passive/RLC Assemblies/RLC (Three-Phase)  port_option=ee.enum.threePhasePort.composite  component_structure=ee.enum.rlc.structure.C  R=1 Ohm  L=1e-3 H  C=2.0278e-08 F  R_parasitic=1 Ohm  G_parasitic=0 1/Ohm  IL_specify=off  IL_priority=High  IL=[0, 0, 0] A  IL_nominal_specify=off  IL_nominal_value=1  IL_nominal_unit=A  VC_specify=off  VC_priority=High  VC=[0, 0, 0] V  VC_nominal_specify=off  VC_nominal_value=1  VC_nominal_unit=V
  Br_4_5_C1_G : ee_lib/Connectors & References/Grounded Neutral (Three-Phase)  port_option=ee.enum.threePhasePort.composite
  Br_4_5_C2 : ee_lib/Passive/RLC Assemblies/RLC (Three-Phase)  port_option=ee.enum.threePhasePort.composite  component_structure=ee.enum.rlc.structure.C  R=1 Ohm  L=1e-3 H  C=2.0278e-08 F  R_parasitic=1 Ohm  G_parasitic=0 1/Ohm  IL_specify=off  IL_priority=High  IL=[0, 0, 0] A  IL_nominal_specify=off  IL_nominal_value=1  IL_nominal_unit=A  VC_specify=off  VC_priority=High  VC=[0, 0, 0] V  VC_nominal_specify=off  VC_nominal_value=1  VC_nominal_unit=V
  Br_4_5_C2_G : ee_lib/Connectors & References/Grounded Neutral (Three-Phase)  port_option=ee.enum.threePhasePort.composite
  Br_4_5_RL : ee_lib/Passive/RLC Assemblies/RLC (Three-Phase)  port_option=ee.enum.threePhasePort.composite  component_structure=ee.enum.rlc.structure.SeriesRL  R=1.5711 Ohm  L=0.050011 H  C=1e-6 F  R_parasitic=0 Ohm  G_parasitic=0 1/Ohm  IL_specify=off  IL_priority=High  IL=[0, 0, 0] A  IL_nominal_specify=off  IL_nominal_value=1  IL_nominal_unit=A  VC_specify=off  VC_priority=High  VC=[0, 0, 0] V  VC_nominal_specify=off  VC_nominal_value=1  VC_nominal_unit=V
  Load_Bus3 : ee_lib/Passive/RLC Assemblies/Wye-Connected Load  port_option=ee.enum.threePhasePort.composite  parameterization=ee.enum.rlc.parameterization.ratedpower  component_structure=ee.enum.rlc.structure.R  component_structure_PQ=ee.enum.rlc.structure.R  R=1 Ohm  L=1e-3 H  C=1e-6 F  VRated=230e3 V  FRated=50 Hz  P=300000000 W  Qpos=98610000 A*V  Qneg=-1e2 A*V  R_parasitic=0 Ohm  G_parasitic=0 1/Ohm  R_parasitic_PQ=0 Ohm  G_parasitic_PQ=0 1/Ohm  Vmag0=24e3 V  Vang0=0 deg  Freq0=60 Hz  IL_specify=off  IL_priority=High  IL=[0, 0, 0] A  IL_nominal_specify=off  IL_nominal_value=1  IL_nominal_unit=A  VC_specify=off  VC_priority=High  VC=[0, 0, 0] V  VC_nominal_specify=off  VC_nominal_value=1  VC_nominal_unit=V
  Load_Bus3_N : fl_lib/Electrical/Electrical Elements/Electrical Reference
  Load_Bus4 : ee_lib/Passive/RLC Assemblies/Wye-Connected Load  port_option=ee.enum.threePhasePort.composite  parameterization=ee.enum.rlc.parameterization.ratedpower  component_structure=ee.enum.rlc.structure.R  component_structure_PQ=ee.enum.rlc.structure.R  R=1 Ohm  L=1e-3 H  C=1e-6 F  VRated=230e3 V  FRated=50 Hz  P=400000000 W  Qpos=131470000 A*V  Qneg=-1e2 A*V  R_parasitic=0 Ohm  G_parasitic=0 1/Ohm  R_parasitic_PQ=0 Ohm  G_parasitic_PQ=0 1/Ohm  Vmag0=24e3 V  Vang0=0 deg  Freq0=60 Hz  IL_specify=off  IL_priority=High  IL=[0, 0, 0] A  IL_nominal_specify=off  IL_nominal_value=1  IL_nominal_unit=A  VC_specify=off  VC_priority=High  VC=[0, 0, 0] V  VC_nominal_specify=off  VC_nominal_value=1  VC_nominal_unit=V
  Load_Bus4_N : fl_lib/Electrical/Electrical Elements/Electrical Reference
  SM_Bus1 : Subsystem
  SM_Bus3 : Subsystem
  SM_Bus5 : Subsystem
  Slack_Bus4 : ee_lib/Sources/Voltage Source (Three-Phase)  vline_rms=230e3 V  shift=0 deg  freq=50 Hz  impedance_option=0  SShortCircuit=1e6 A*V  XR=15  R=0.01 Ohm  L=3.97e-4 H  harmonic_option=0  harmonic_orders=[5, 7, 11, 13]  harmonic_ratios=[.1, .1, .1, .1]  G_parasitic=0 1/Ohm  I_specify=off  I_priority=None  I=[0, 0, 0] A  I_nominal_specify=off  I_nominal_value=1  I_nominal_unit=A
  Slack_Bus4_N : fl_lib/Electrical/Electrical Elements/Electrical Reference
  Elec_PCC_230kV : PMIOPort  Side=Left
  connections:
  Slack_Bus4/LConn1 -- Slack_Bus4_N/LConn1
  Load_Bus3/RConn1 -- Load_Bus3_N/LConn1
  Load_Bus4/RConn1 -- Load_Bus4_N/LConn1
  Br_1_2_C1/RConn1 -- Br_1_2_C1_G/LConn1
  Br_1_2_C2/RConn1 -- Br_1_2_C2_G/LConn1
  Br_1_4_C1/RConn1 -- Br_1_4_C1_G/LConn1
  Br_1_4_C2/RConn1 -- Br_1_4_C2_G/LConn1
  Br_1_5_C1/RConn1 -- Br_1_5_C1_G/LConn1
  Br_1_5_C2/RConn1 -- Br_1_5_C2_G/LConn1
  Br_1_5_RL/LConn1 -- Br_1_5_C1/LConn1 -- SM_Bus1/RConn1 -- Br_1_2_C1/LConn1 -- Br_1_2_RL/LConn1 -- Br_1_4_C1/LConn1 -- Br_1_4_RL/LConn1
  Br_2_3_C1/RConn1 -- Br_2_3_C1_G/LConn1
  Br_2_3_C2/RConn1 -- Br_2_3_C2_G/LConn1
  Br_2_3_RL/LConn1 -- Br_2_3_C1/LConn1 -- Elec_PCC_230kV/RConn1 -- Br_1_2_C2/LConn1 -- Br_1_2_RL/RConn1
  Br_3_4_C1/RConn1 -- Br_3_4_C1_G/LConn1
  Br_3_4_C2/RConn1 -- Br_3_4_C2_G/LConn1
  Br_3_4_RL/LConn1 -- Br_3_4_C1/LConn1 -- SM_Bus3/RConn1 -- Br_2_3_C2/LConn1 -- Br_2_3_RL/RConn1 -- Load_Bus3/LConn1
  Br_4_5_C1/RConn1 -- Br_4_5_C1_G/LConn1
  Br_4_5_C2/RConn1 -- Br_4_5_C2_G/LConn1
  Br_4_5_RL/LConn1 -- Br_4_5_C1/LConn1 -- Slack_Bus4/RConn1 -- Br_1_4_C2/LConn1 -- Br_1_4_RL/RConn1 -- Br_3_4_C2/LConn1 -- Br_3_4_RL/RConn1 -- Load_Bus4/LConn1
  Br_4_5_RL/RConn1 -- Br_4_5_C2/LConn1 -- SM_Bus5/RConn1 -- Br_1_5_C2/LConn1 -- Br_1_5_RL/RConn1

== system microgrid_case5/Wind ==
  In_v_wind_ms : Inport
  Gnd : fl_lib/Electrical/Electrical Elements/Electrical Reference
  I_S2PS : nesl_utility/Simulink-PS Converter  PhysicalDomain=network_engine_domain  SubClassName=ps_input  LeftPortType=input  RightPortType=output  PseudoPeriodic=off  Frequencies=[]  NoiseDistribution=none  NoiseParameters=[]  Unit=A  AffineConversion=off  FilteringAndDerivatives=filter  SimscapeFilterOrder=1  InputFilterTimeConstant=1e-4  UdotUserProvided=0
  I_delay : UnitDelay  SampleTime=5e-05
  V_dc_sens : fl_lib/Electrical/Electrical Sensors/Voltage Sensor
  Vdc_PS2S : nesl_utility/PS-Simulink Converter  PhysicalDomain=network_engine_domain  SubClassName=ps_output  LeftPortType=input  RightPortType=output  PseudoPeriodic=off  Frequencies=[]  VectorFormat=inherit  Unit=V  AffineConversion=off
  Wind_CCS : fl_lib/Electrical/Electrical Sources/Controlled Current Source
  dcdc_ctrl : MATLAB Function  TreatAsAtomicUnit=on
  wind_turbine : MATLAB Function  TreatAsAtomicUnit=on
  Elec_DC_out : PMIOPort  Side=Left
  Out_P_wind_MW : Outport
  Out_v_wind_ms : Outport  Port=2
  Out_Cp : Outport  Port=3
  wires:
  In_v_wind_ms/1 -> Out_v_wind_ms/1, wind_turbine/1(v)
  wind_turbine/2(Cp) -> Out_Cp/1
  wind_turbine/1(P_turb_W) -> dcdc_ctrl/1(P_turb_W)
  Vdc_PS2S/1 -> dcdc_ctrl/2(V_dc_V)
  dcdc_ctrl/2(P_bus_MW) -> Out_P_wind_MW/1
  dcdc_ctrl/1(I_cmd_A) -> I_delay/1
  I_delay/1 -> I_S2PS/1
  connections:
  V_dc_sens/LConn1 -- Elec_DC_out/RConn1 -- Wind_CCS/LConn1
  Gnd/LConn1 -- V_dc_sens/RConn2 -- Wind_CCS/RConn2
  V_dc_sens/RConn1 -- Vdc_PS2S/LConn1
  I_S2PS/RConn1 -- Wind_CCS/RConn1

== system microgrid_case5/MicrogridACBus/ZigZagGrounding ==
  EarthingXFMR : ee_lib/Passive/Transformers/Earthing Transformer  SRated=2000000 A*V  VRated=33000 V  FRated=50 Hz  Unit=ee.enum.unit.pu  pu_Rw=0.01  pu_Xl=0.3  pu_Rm=500  pu_Xm=500  si_Rw=0.0576 Ohm  si_Ll=1.728 H  si_Rm=2880 Ohm  si_Lm=2880 H  i1_specify=off  i1_priority=None  i1=[0, 0, 0] A  i1_nominal_specify=off  i1_nominal_value=1  i1_nominal_unit=A  phi1_specify=off  phi1_priority=None  phi1=[0, 0, 0] Wb  phi1_nominal_specify=off  phi1_nominal_value=1  phi1_nominal_unit=Wb
  Gnd : fl_lib/Electrical/Electrical Elements/Electrical Reference
  I_neutral : fl_lib/Electrical/Electrical Sensors/Current Sensor
  In_PS2S : nesl_utility/PS-Simulink Converter  PhysicalDomain=network_engine_domain  SubClassName=ps_output  LeftPortType=input  RightPortType=output  PseudoPeriodic=off  Frequencies=[]  VectorFormat=inherit  Unit=A  AffineConversion=off
  NGR : ee_lib/Passive/Resistor  R=47 Ohm  enable_R_tol=ee.enum.toleranceApplication.none  R_tol=5  tol_distribution=ee.enum.toleranceDistribution.uniform  nSigma=4  enable_operating_limits=ee.enum.enable.no  operating_limit_action=ee.enum.passive.reportOpLim.warn  power_rating=1 W  max_working_voltage=100 V  noise_mode=ee.enum.sources.noise.Disabled  Tdevice=25 degC  sample_time=1e-3 s  repeatability=ee.enum.ic.repeatability.notRepeatable  user_seed=0  auto_seed=3499211588  power_derating_T1=70 degC  power_derating_T2=155 degC  operating_temperature_range_vec=[-50, 150] degC  alpha=3.93e-3 1/K  Tmeas=25 degC  thermal_mass=100 J/K  temperature_specify=off  temperature_priority=High  temperature=298.15 K  temperature_nominal_specify=off  temperature_nominal_value=1  temperature_nominal_unit=K
  Elec_AC_33kV : PMIOPort  Side=Left
  Out_I_neutral_A : Outport
  wires:
  In_PS2S/1 -> Out_I_neutral_A/1
  connections:
  Elec_AC_33kV/RConn1 -- EarthingXFMR/LConn1
  EarthingXFMR/RConn1 -- I_neutral/LConn1
  I_neutral/RConn2 -- NGR/LConn1
  NGR/RConn1 -- Gnd/LConn1
  I_neutral/RConn1 -- In_PS2S/LConn1

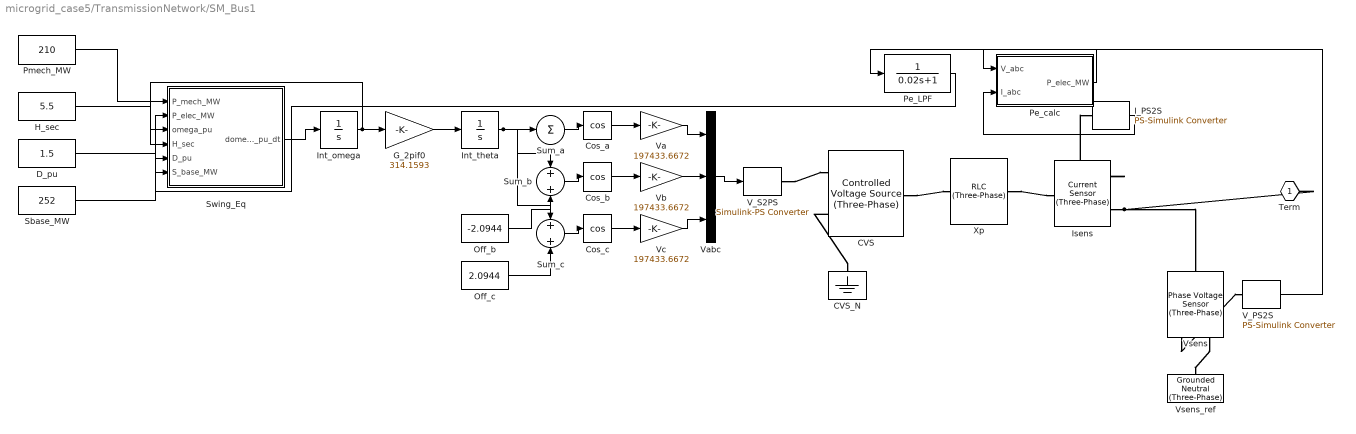
== system microgrid_case5/TransmissionNetwork/SM_Bus1 ==
  CVS : ee_lib/Sources/Controlled Voltage Source (Three-Phase)  input_option=ee.enum.inputType.instantaneous  FRated=60 Hz
  CVS_N : fl_lib/Electrical/Electrical Elements/Electrical Reference
  Cos_a : Trigonometry  Operator=cos
  Cos_b : Trigonometry  Operator=cos
  Cos_c : Trigonometry  Operator=cos
  D_pu : Constant  Value=1.5
  G_2pif0 : Gain  Gain=314.1593
  H_sec : Constant  Value=5.5
  I_PS2S : nesl_utility/PS-Simulink Converter  PhysicalDomain=network_engine_domain  SubClassName=ps_output  LeftPortType=input  RightPortType=output  PseudoPeriodic=off  Frequencies=[]  VectorFormat=inherit  Unit=inherit  AffineConversion=off
  Int_omega : Integrator  InitialCondition=1.0
  Int_theta : Integrator  InitialCondition=0.25661
  Isens : ee_lib/Sensors & Transducers/Current Sensor (Three-Phase)  port_option=ee.enum.threePhasePort.composite
  Off_b : Constant  Value=-2.0944
  Off_c : Constant  Value=2.0944
  Pe_LPF : TransferFcn  Denominator=[0.02 1]
  Pe_calc : MATLAB Function  TreatAsAtomicUnit=on
  Pmech_MW : Constant  Value=210
  Sbase_MW : Constant  Value=252
  Sum_a : Sum  Inputs=+
  Sum_b : Sum
  Sum_c : Sum
  Swing_Eq : MATLAB Function  TreatAsAtomicUnit=on
  V_PS2S : nesl_utility/PS-Simulink Converter  PhysicalDomain=network_engine_domain  SubClassName=ps_output  LeftPortType=input  RightPortType=output  PseudoPeriodic=off  Frequencies=[]  VectorFormat=inherit  Unit=inherit  AffineConversion=off
  V_S2PS : nesl_utility/Simulink-PS Converter  PhysicalDomain=network_engine_domain  SubClassName=ps_input  LeftPortType=input  RightPortType=output  PseudoPeriodic=off  Frequencies=[]  NoiseDistribution=none  NoiseParameters=[]  Unit=V  AffineConversion=off  FilteringAndDerivatives=filter  SimscapeFilterOrder=1  InputFilterTimeConstant=1e-4  UdotUserProvided=0
  Va : Gain  Gain=197433.6672
  Vabc : Mux  Inputs=3
  Vb : Gain  Gain=197433.6672
  Vc : Gain  Gain=197433.6672
  Vsens : ee_lib/Sensors & Transducers/Phase Voltage Sensor (Three-Phase)  port_option=ee.enum.threePhasePort.composite
  Vsens_ref : ee_lib/Connectors & References/Grounded Neutral (Three-Phase)  port_option=ee.enum.threePhasePort.composite
  Xp : ee_lib/Passive/RLC Assemblies/RLC (Three-Phase)  port_option=ee.enum.threePhasePort.composite  component_structure=ee.enum.rlc.structure.SeriesRL  R=0.001 Ohm  L=0.16705 H  C=1e-6 F  R_parasitic=0 Ohm  G_parasitic=0 1/Ohm  IL_specify=off  IL_priority=High  IL=[0, 0, 0] A  IL_nominal_specify=off  IL_nominal_value=1  IL_nominal_unit=A  VC_specify=off  VC_priority=High  VC=[0, 0, 0] V  VC_nominal_specify=off  VC_nominal_value=1  VC_nominal_unit=V
  Term : PMIOPort  Side=Right
  wires:
  V_PS2S/1 -> Pe_calc/1(V_abc)
  I_PS2S/1 -> Pe_calc/2(I_abc)
  Pe_calc/1(P_elec_MW) -> Pe_LPF/1
  Pmech_MW/1 -> Swing_Eq/1(P_mech_MW)
  Pe_LPF/1 -> Swing_Eq/2(P_elec_MW)
  Int_omega/1 -> Swing_Eq/3(omega_pu), G_2pif0/1
  H_sec/1 -> Swing_Eq/4(H_sec)
  D_pu/1 -> Swing_Eq/5(D_pu)
  Sbase_MW/1 -> Swing_Eq/6(S_base_MW)
  Swing_Eq/1(domega_pu_dt) -> Int_omega/1
  G_2pif0/1 -> Int_theta/1
  Int_theta/1 -> Sum_a/1, Sum_b/1, Sum_c/1
  Off_b/1 -> Sum_b/2
  Off_c/1 -> Sum_c/2
  Sum_a/1 -> Cos_a/1
  Sum_b/1 -> Cos_b/1
  Sum_c/1 -> Cos_c/1
  Cos_a/1 -> Va/1
  Cos_b/1 -> Vb/1
  Cos_c/1 -> Vc/1
  Va/1 -> Vabc/1
  Vb/1 -> Vabc/2
  Vc/1 -> Vabc/3
  Vabc/1 -> V_S2PS/1
  connections:
  CVS/LConn2 -- CVS_N/LConn1
  V_S2PS/RConn1 -- CVS/LConn1
  CVS/RConn1 -- Xp/LConn1
  Xp/RConn1 -- Isens/LConn1
  Term/RConn1 -- Isens/RConn2 -- Vsens/LConn1
  Vsens/RConn2 -- Vsens_ref/LConn1
  Isens/RConn1 -- I_PS2S/LConn1
  Vsens/RConn1 -- V_PS2S/LConn1
